simulink model "mdlFloat"  (Simulink 5.2)
settings: Solver=FixedStepDiscrete  StartTime=0.0  StopTime=inf  RelTol=1e-3
PreLoadFcn:
  | mdlData;
values from neighbouring files (symbols this model uses):
  exp_mapE_X = single([-2;-1.5e+000;-1;-5e-001;0;5e-001;1;1.5e+000;2;2.5e+000;3;3.5e+000;4;4.5e+000;5;5.5e+000;6;6.5e+000;7;7.5e+000;8;8.5e+000;9;9.5e+000;10])    [mdlData.m]
  exp_mapE_Y = single([1.353352832366127e-001;2.2313016014842982e-001;3.6787944117144233e-001;6.065306597126334e-001;1;1.6487212707001282e+000;2.7182818284590455e+000;4.4816890703380645e+000;7.38905609893065e+000;1.2182493960703473e+001;2.0085536923187668e+001;3.311545195869231e+001;5.4598150033144236e+001;9.001713130052181e+001;1.484131591025766e+002;2.4469193226422038e+002;4.034287934927351e+002;6.651416330443 ...(+176 chars)    [mdlData.m]
  exp_mapU_X = single([-2;3.6210732460021973e+000;5.016105651855469e+000;5.833150863647461e+000;6.412175178527832e+000;6.860101699829102e+000;7.226192474365234e+000;7.535517692565918e+000;7.803262710571289e+000;8.03936767578125e+000;8.250225067138672e+000;8.441097259521484e+000;8.61508560180664e+000;8.775198936462402e+000;8.923519134521484e+000;9.061382293701172e+000;9.190909385681152e+000;9.312210083007813e+000 ...(+142 chars)    [mdlData.m]
  exp_mapU_Y = single([1.353352832366127e-001;3.737766172891453e+001;1.5082280212302192e+002;3.4143279416719156e+002;6.092173974815711e+002;9.534640296894547e+002;1.374977263551756e+003;1.8734139602370635e+003;2.448577960082799e+003;3.100651953000505e+003;3.8284873911833256e+003;4.633636497945872e+003;5.514220620782577e+003;6.47173127340932e+003;7.506459042164025e+003;8.616052341195369e+003;9.80756578498257e+003 ...(+190 chars)    [mdlData.m]
  m_sng_01 = [1 2 3; 4 5 6; 7 8 9]    [mdlData.m]
  m_sng_02 = [9 8 7; 6 5 4; 3 2 1]    [mdlData.m]
  map3D_Z = [4 5 6;16 19 20;10 18 23]    [mdlData.m]
  p_sng_01 = 1    [mdlData.m]
  p_sng_02 = 2    [mdlData.m]
  ss_A = [1 2 3; 4 5 6; 7 8 9]    [mdlData.m]
  ss_B = [0;0;1]    [mdlData.m]
  ss_C = [9 8 7; 6 5 4; 3 2 1]    [mdlData.m]
  ss_D = [0.5;0.5;0]    [mdlData.m]
libraries: simulink x8, lib_CATutils_Utilities_DocBlock x4, lib_CATutils_Utilities_RevNoteBlock x3, package_instance x1
settings Model: LastModifiedBy=KagyRA  ExtModeMexFile=no_ext_comm  SaveTime=off  SaveOutput=off  LimitDataPoints=off  ParameterPrecisionLossMsg=none  RTWInlineParameters=on  BooleanDataType=on  ProdHWDeviceType=Microprocessor  RTWSystemTargetFile=cat_ert.tlc  RTWTemplateMakefile=cat_ert_default_tmf  RTWGenerateCodeOnly=on  RTWRetainRTWFile=on  RTWOptions="-aASAP2FileDirectory=\".\" -aCAT_MaxStackSize=\"rtInf\" -aCAT_OVregexp=\"\" -aCadetWinFileDirectory=\".\" -aCatASAP2Config_MeasurementSignalGroups=\"Model_Hierarchy_Only\" -aCatASAP2Config_ModelHierarchyGroups=\"Pruned_Model_Hierarchy\" -aCatASAP2Config_SymbolNamingCompiler=\"A4_(Diab_ELF)\" -aCatCadetWinConfig_CreateArrayParameter=1 -aCatCadetWinConfig_CreateArraySignal=1 -aCatCadetWinConfig_CreateMap=1 -aCatCadetWinConfig_MID=\"0xFF\" -aCatCalToolConfig_ConvertPIDF=0 -aCatCalToolConfig_CreateASAP2=0 -aCatCalToolConfig_CreateCadetWin=0 -aCatCalToolConfig_CreateDebug=0 -aCatCalToolConfig_CreateEMC2=0 -aCatCalToolConfig_CreateGredi=0 -aCatEMC2Config_AppendInstance=1 -aCatEMC2Config_ApplyStaticVarBandAid=0 -aCatEMC2Config_CreateUnnamedVariables=0 -aCatEMC2Config_GenerateMapFile=1 -aCatEMC2Config_GenerateParFile=1 -aCatEMC2Config_GenerateRemapFcnFile=0 -aCatEMC2Config_MangleParameters=\"Add_underscore_h_to_Param_entry\" -aCatEMC2Config_NameGuidelines=\"Short_Name_Valid_in_all_Tools\" -aCatGrediConfig_BinBaseAddress=\"0x2DA000\" -aCatGrediConfig_BinSize=40 -aCatGrediConfig_CANBaudrate=250 -aCatGrediConfig_CROID=\"0x2010000\" -aCatGrediConfig_DTOID=\"0x2020000\" -aCatGrediConfig_ECUType=\"0x022D\" -aCatGrediConfig_MeasurementBaseAddress=\"0x2C0800\" -aCatGrediConfig_NodeID=\"0x0001\" -aCatGrediConfig_SampleInterval=20 -aCatGrediConfig_TID=1 -aCat_CheckForScopeDisplayBlocks=0 -aCat_RedExclmPreventCodeGen=0 -aCat_SkipEMC2GeneratedFiles=0 -aCombineOutputUpdateFcns=1 -aConfigSourceFileDirectory=\".\" -aEMC2SourceFileDirectory=\".\" -aERTCreateCustomFiles=1 -aERTCustomFileBanners=0 -aERTCustomFileTemplate=\"example_file_process.tlc\" -aERTHdrFileBannerTemplate=\"example_banner.tlc\" -aERTSrcFileBannerTemplate=\"example_banner.tlc\" -aEnforceIntegerDowncast=1 -aExtMode=0 -aExtModeTesting=0 -aFixPtUtilType=\"macro\" -aFoldNonRolledExpr=1 -aForceParamTrailComments=0 -aGenFloatMathFcnCalls=\"ANSI_C\" -aGenerateASAP2=0 -aGenerateComments=1 -aGenerateErtSFunction=0 -aGeneratePackageArchCode=\"ModelCodeAndPackageObjectFile\" -aGenerateReport=0 -aGenerateSampleERTMain=0 -aGrediFileDirectory=\".\" -aIgnoreCustomStorageClasses=0 -aIncDataTypeInIds=0 -aIncHierarchyInIds=0 -aIncludeMdlTerminateFcn=1 -aInitFltsAndDblsToZero=1 -aInlineInvariantSignals=0 -aInlineParameters=1 -aInlinedParameterPlacement=\"NonHierarchical\" -aInlinedPrmAccess=\"Literals\" -aInsertBlockDesc=0 -aLocalBlockOutputs=1 -aMapIncludeFileDirectory=\".\" -aMapSourceFileDirectory=\".\" -aMatFileLogging=0 -aMaxRTWIdLen=31 -aMultiInstanceERTCode=1 -aMultiInstanceErrorCode=\"None\" -aPackageIncludeFileDirectory=\".\" -aPackageSourceFileDirectory=\".\" -aPrefixModelToSubsysFcnNames=1 -aPurelyIntegerCode=0 -aRTWVerbose=1 -aRfdDevelopTableStructFileName=\"<DevelopTableStructFileName>\" -aRfdDevelopTableStructName=\"<DevelopTableStructName>\" -aRfdIncludeFileDirectory=\".\" -aRfdSourceFileDirectory=\".\" -aRollThreshold=5 -aRootIOStructures=0 -aShowEliminatedStatements=0 -aSpecialFilesAndDirectories=\"\" -aSuppressErrorStatus=1 -aTargetOS=\"None\" -aTuneIncludeFileDirectory=\".\" -aZeroExternalMemoryAtStartup=0 -aZeroInternalMemoryAtStartup=1"

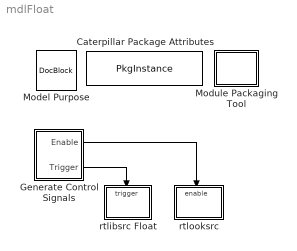
== system mdlFloat ==
  Caterpillar Package Attributes : package_instance/PkgInstance  pkgName=mdlFloat  InitTaskTag=SSS_TID_INIT  availModelRates={ '1.000', 'SSS_TID_1005MSEC'; '0.12', 'SSS_TID_120MSEC'; }
  Generate Control Signals : Subsystem
  Model Purpose : lib_CATutils_Utilities_DocBlock/DocBlock  isHTML=off
  Module Packaging Tool : Subsystem  Description=MPM
      settings: AttributesFormatString=Module\nPackaging\nTool\n  CopyFcn=mcb('mdlFloat')  ModelCloseFcn=mpm_callback('MPTClose',[])  PreSaveFcn=set_param(gcb, 'CopyFcn', ['mcb(''', bdroot, ''')']);  OpenFcn=mpm_gui_options(bdroot)
      mask Type: ModulePackagingTool
      mask Description: This is the Module Packaging Tool
      mask Display: image(imread('mpm_icon.bmp','bmp'))
  rtlibsrc Float : Subsystem
  rtlooksrc : Subsystem
  wires:
  Generate Control Signals/2(Trigger) -> rtlibsrc Float/Trigger
  Generate Control Signals/1(Enable) -> rtlooksrc/Enable

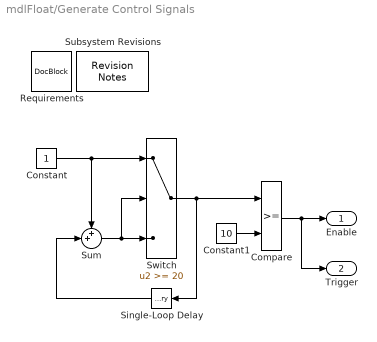
== system mdlFloat/Generate Control Signals ==
  Compare : RelationalOperator  ShowAdditionalParam=on  LogicOutDataTypeMode=Specify via dialog  LogicDataType=float('single')  InputSameDT=on
  Constant : Constant  ShowAdditionalParam=on  OutDataTypeMode=single  SampleTime=1
  Constant1 : Constant  Value=10  ShowAdditionalParam=on
  Requirements : lib_CATutils_Utilities_DocBlock/DocBlock  isHTML=off
  Single-Loop Delay : Memory  Orientation=left  InheritSampleTime=on
  Subsystem Revisions : lib_CATutils_Utilities_RevNoteBlock/Revision Notes  data=struct('User','---','Date',730486,'Revision','---')
  Sum : Sum  Inputs=++|  SaturateOnIntegerOverflow=on  InputSameDT=on
  Switch : Switch  Threshold=20  SaturateOnIntegerOverflow=on  InputSameDT=on
  Enable : Outport
  Trigger : Outport  Port=2
  wires:
  Constant/1 -> Switch/1, Sum/1
  Sum/1 -> Switch/3, Switch/2
  Switch/1 -> Single-Loop Delay/1, Compare/1
  Single-Loop Delay/1 -> Sum/2
  Constant1/1 -> Compare/2
  Compare/1 -> Enable/1, Trigger/1

== system mdlFloat/Module Packaging Tool ==
  Subsystem : Subsystem

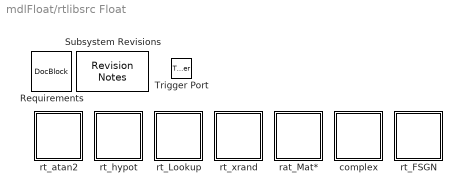
== system mdlFloat/rtlibsrc Float ==
  Trigger Port : TriggerPort  TriggerType=either
  Requirements : lib_CATutils_Utilities_DocBlock/DocBlock  isHTML=off
  Subsystem Revisions : lib_CATutils_Utilities_RevNoteBlock/Revision Notes  data=struct('User','---','Date',730486,'Revision','---')
  complex : Subsystem
  rat_Mat* : Subsystem
  rt_FSGN : Subsystem
  rt_Lookup : Subsystem
  rt_atan2 : Subsystem
  rt_hypot : Subsystem
  rt_xrand : Subsystem

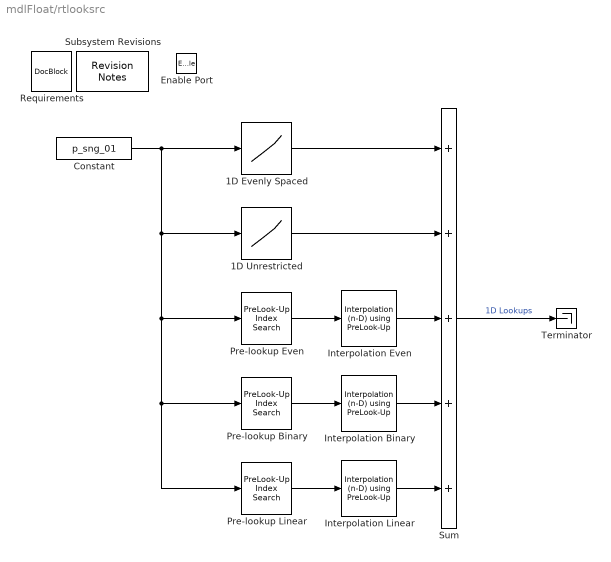
== system mdlFloat/rtlooksrc ==
  Enable Port : EnablePort  StatesWhenEnabling=reset
  1D Evenly Spaced : Lookup  InputValues=exp_mapE_X  OutputValues=exp_mapE_Y  ShowAdditionalParam=on  LookUpMeth=Interpolation-Use End Values  SaturateOnIntegerOverflow=on
  1D Unrestricted : Lookup  InputValues=exp_mapU_X  OutputValues=exp_mapU_Y  ShowAdditionalParam=on  LookUpMeth=Interpolation-Use End Values  SaturateOnIntegerOverflow=on
  Constant : Constant  Value=p_sng_01  ShowAdditionalParam=on  OutDataTypeMode=single
  Interpolation Binary : simulink/Look-Up Tables/Interpolation (n-D) using PreLook-Up  numDimsPopupSelect=1  explicitNumDims=2  table=exp_mapU_Y  interpMethod=Linear  extrapMethod=None - Clip  rangeErrorMode=None
  Interpolation Even : simulink/Look-Up Tables/Interpolation (n-D) using PreLook-Up  numDimsPopupSelect=1  explicitNumDims=2  table=exp_mapE_Y  interpMethod=Linear  extrapMethod=None - Clip  rangeErrorMode=None
  Interpolation Linear : simulink/Look-Up Tables/Interpolation (n-D) using PreLook-Up  numDimsPopupSelect=1  explicitNumDims=2  table=exp_mapU_Y  interpMethod=Linear  extrapMethod=None - Clip  rangeErrorMode=None
  Pre-lookup Binary : simulink/Look-Up Tables/PreLook-Up Index Search  bpData=exp_mapU_X  searchMode=Binary Search  cacheBpFlag=off  outputFlag=off  extrapMode=Clip to Range  rangeErrorMode=None
  Pre-lookup Even : simulink/Look-Up Tables/PreLook-Up Index Search  bpData=exp_mapE_X  searchMode=Evenly Spaced Points  cacheBpFlag=on  outputFlag=off  extrapMode=Clip to Range  rangeErrorMode=None
  Pre-lookup Linear : simulink/Look-Up Tables/PreLook-Up Index Search  bpData=exp_mapU_X  searchMode=Linear Search  cacheBpFlag=on  outputFlag=off  extrapMode=Clip to Range  rangeErrorMode=None
  Requirements : lib_CATutils_Utilities_DocBlock/DocBlock  isHTML=off
  Subsystem Revisions : lib_CATutils_Utilities_RevNoteBlock/Revision Notes  data=struct('User','---','Date',730486,'Revision','---')
  Sum : Sum  Inputs=5  ShowAdditionalParam=on  SaturateOnIntegerOverflow=on  InputSameDT=on
  Terminator : Terminator
  wires:
  Constant/1 -> 1D Evenly Spaced/1, 1D Unrestricted/1, Pre-lookup Binary/1, Pre-lookup Linear/1, Pre-lookup Even/1
  Sum/1 -> Terminator/1  "1D Lookups"
  Pre-lookup Even/1 -> Interpolation Even/1
  Pre-lookup Binary/1 -> Interpolation Binary/1
  Pre-lookup Linear/1 -> Interpolation Linear/1
  1D Evenly Spaced/1 -> Sum/1
  1D Unrestricted/1 -> Sum/2
  Interpolation Even/1 -> Sum/3
  Interpolation Binary/1 -> Sum/4
  Interpolation Linear/1 -> Sum/5

== system mdlFloat/Module Packaging Tool/Subsystem ==

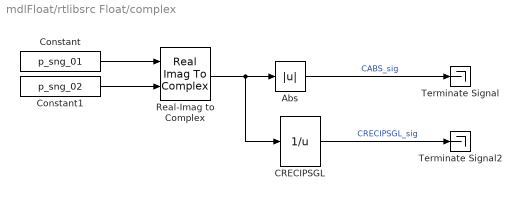
== system mdlFloat/rtlibsrc Float/complex ==
  Abs : Abs  SaturateOnIntegerOverflow=on
  CRECIPSGL : Math  Operator=reciprocal
  Constant : Constant  Value=p_sng_01  ShowAdditionalParam=on  OutDataTypeMode=single
  Constant1 : Constant  Value=p_sng_02  ShowAdditionalParam=on
  Real-Imag to Complex : RealImagToComplex
  Terminate Signal : Terminator
  Terminate Signal2 : Terminator
  wires:
  Constant1/1 -> Real-Imag to Complex/2
  Constant/1 -> Real-Imag to Complex/1
  Real-Imag to Complex/1 -> Abs/1, CRECIPSGL/1
  Abs/1 -> Terminate Signal/1  "CABS_sig"
  CRECIPSGL/1 -> Terminate Signal2/1  "CRECIPSGL_sig"

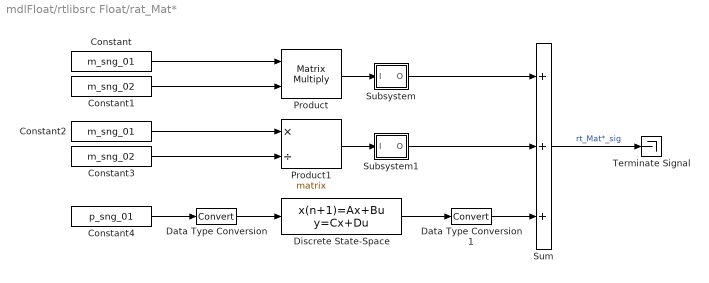
== system mdlFloat/rtlibsrc Float/rat_Mat* ==
  Constant : Constant  Value=m_sng_01  VectorParams1D=off  ShowAdditionalParam=on  OutDataTypeMode=single
  Constant1 : Constant  Value=m_sng_02  VectorParams1D=off  ShowAdditionalParam=on  OutDataTypeMode=single
  Constant2 : Constant  Value=m_sng_01  VectorParams1D=off  ShowAdditionalParam=on  OutDataTypeMode=single
  Constant3 : Constant  Value=m_sng_02  VectorParams1D=off  ShowAdditionalParam=on  OutDataTypeMode=single
  Constant4 : Constant  Value=p_sng_01  ShowAdditionalParam=on  OutDataTypeMode=single
  Data Type Conversion : DataTypeConversion  DataType=double  SaturateOnIntegerOverflow=on
  Data Type Conversion1 : DataTypeConversion  DataType=single  SaturateOnIntegerOverflow=on
  Discrete State-Space : DiscreteStateSpace  A=ss_A  B=ss_B  C=ss_C  D=ss_D  SampleTime=-1
  Product : Product  Multiplication=Matrix(*)  ShowAdditionalParam=on  SaturateOnIntegerOverflow=on  InputSameDT=on
  Product1 : Product  Inputs=*/  Multiplication=Matrix(*)  ShowAdditionalParam=on  SaturateOnIntegerOverflow=on  InputSameDT=on
  Subsystem : Subsystem
  Subsystem1 : Subsystem
  Sum : Sum  Inputs=3  ShowAdditionalParam=on  SaturateOnIntegerOverflow=on  InputSameDT=on
  Terminate Signal : Terminator
  wires:
  Sum/1 -> Terminate Signal/1  "rt_Mat*_sig"
  Constant/1 -> Product/1
  Constant1/1 -> Product/2
  Constant2/1 -> Product1/1
  Constant3/1 -> Product1/2
  Constant4/1 -> Data Type Conversion/1
  Product/1 -> Subsystem/1(I)
  Product1/1 -> Subsystem1/1(I)
  Discrete State-Space/1 -> Data Type Conversion1/1
  Subsystem/1(O) -> Sum/1
  Subsystem1/1(O) -> Sum/2
  Data Type Conversion/1 -> Discrete State-Space/1
  Data Type Conversion1/1 -> Sum/3

== system mdlFloat/rtlibsrc Float/rt_FSGN ==
  Constant : Constant  Value=p_sng_01  ShowAdditionalParam=on  OutDataTypeMode=single
  Sign : Signum
  Terminate Signal : Terminator
  wires:
  Sign/1 -> Terminate Signal/1  "rt_FSGN_sig"
  Constant/1 -> Sign/1

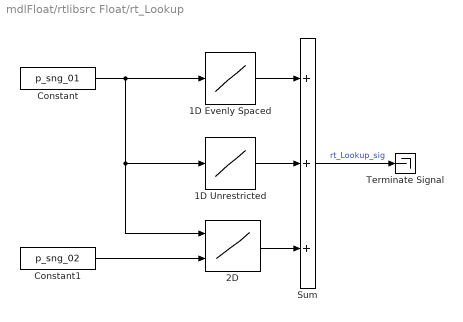
== system mdlFloat/rtlibsrc Float/rt_Lookup ==
  1D Evenly Spaced : Lookup  InputValues=exp_mapE_X  OutputValues=exp_mapE_Y  ShowAdditionalParam=on  LookUpMeth=Interpolation-Use End Values  SaturateOnIntegerOverflow=on
  1D Unrestricted : Lookup  InputValues=exp_mapU_X  OutputValues=exp_mapU_Y  ShowAdditionalParam=on  LookUpMeth=Interpolation-Use End Values  SaturateOnIntegerOverflow=on
  2D : Lookup2D  RowIndex=map3D_X  ColumnIndex=map3D_Y  OutputValues=map3D_Z  ShowAdditionalParam=on  LookUpMeth=Interpolation-Use End Values  SaturateOnIntegerOverflow=on  InputSameDT=on
  Constant : Constant  Value=p_sng_01  ShowAdditionalParam=on  OutDataTypeMode=single
  Constant1 : Constant  Value=p_sng_02  ShowAdditionalParam=on  OutDataTypeMode=single
  Sum : Sum  Inputs=3  ShowAdditionalParam=on  SaturateOnIntegerOverflow=on  InputSameDT=on
  Terminate Signal : Terminator
  wires:
  Sum/1 -> Terminate Signal/1  "rt_Lookup_sig"
  Constant/1 -> 1D Evenly Spaced/1, 1D Unrestricted/1, 2D/1
  1D Evenly Spaced/1 -> Sum/1
  1D Unrestricted/1 -> Sum/2
  Constant1/1 -> 2D/2
  2D/1 -> Sum/3

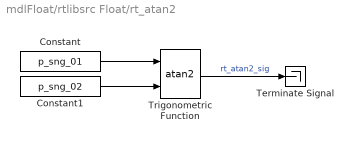
== system mdlFloat/rtlibsrc Float/rt_atan2 ==
  Constant : Constant  Value=p_sng_01  ShowAdditionalParam=on  OutDataTypeMode=single
  Constant1 : Constant  Value=p_sng_02  ShowAdditionalParam=on
  Terminate Signal : Terminator
  Trigonometric Function : Trigonometry  Operator=atan2
  wires:
  Constant/1 -> Trigonometric Function/1
  Trigonometric Function/1 -> Terminate Signal/1  "rt_atan2_sig"
  Constant1/1 -> Trigonometric Function/2

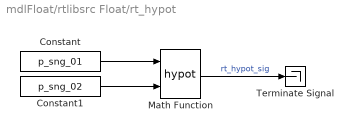
== system mdlFloat/rtlibsrc Float/rt_hypot ==
  Constant : Constant  Value=p_sng_01  ShowAdditionalParam=on  OutDataTypeMode=single
  Constant1 : Constant  Value=p_sng_02  ShowAdditionalParam=on
  Math Function : Math  Operator=hypot
  Terminate Signal : Terminator
  wires:
  Constant1/1 -> Math Function/2
  Math Function/1 -> Terminate Signal/1  "rt_hypot_sig"
  Constant/1 -> Math Function/1

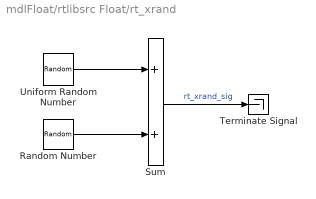
== system mdlFloat/rtlibsrc Float/rt_xrand ==
  Random Number : RandomNumber  Mean=2
  Sum : Sum  Inputs=2  ShowAdditionalParam=on  SaturateOnIntegerOverflow=on  InputSameDT=on
  Terminate Signal : Terminator
  Uniform Random Number : UniformRandomNumber
  wires:
  Sum/1 -> Terminate Signal/1  "rt_xrand_sig"
  Uniform Random Number/1 -> Sum/1
  Random Number/1 -> Sum/2

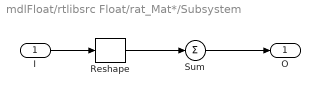
== system mdlFloat/rtlibsrc Float/rat_Mat*/Subsystem ==
  I : Inport
  Reshape : simulink/Math Operations/Reshape  OutputDimensionality=1-D array  OutputDimensions=[1,1]
  Sum : Sum  Inputs=1  ShowAdditionalParam=on  SaturateOnIntegerOverflow=on  InputSameDT=on
  O : Outport
  wires:
  I/1 -> Reshape/1
  Reshape/1 -> Sum/1
  Sum/1 -> O/1

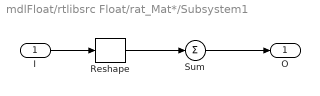
== system mdlFloat/rtlibsrc Float/rat_Mat*/Subsystem1 ==
  I : Inport
  Reshape : simulink/Math Operations/Reshape  OutputDimensionality=1-D array  OutputDimensions=[1,1]
  Sum : Sum  Inputs=1  ShowAdditionalParam=on  SaturateOnIntegerOverflow=on  InputSameDT=on
  O : Outport
  wires:
  Sum/1 -> O/1
  Reshape/1 -> Sum/1
  I/1 -> Reshape/1
